simulink model "Q2_model"  (R2019a)
settings: Solver=VariableStepAuto  StartTime=0.0  StopTime=3  RelTol=1e-3
libraries: dspsigops x3
settings Model: Creator=Admin  LastModifiedBy=Admin

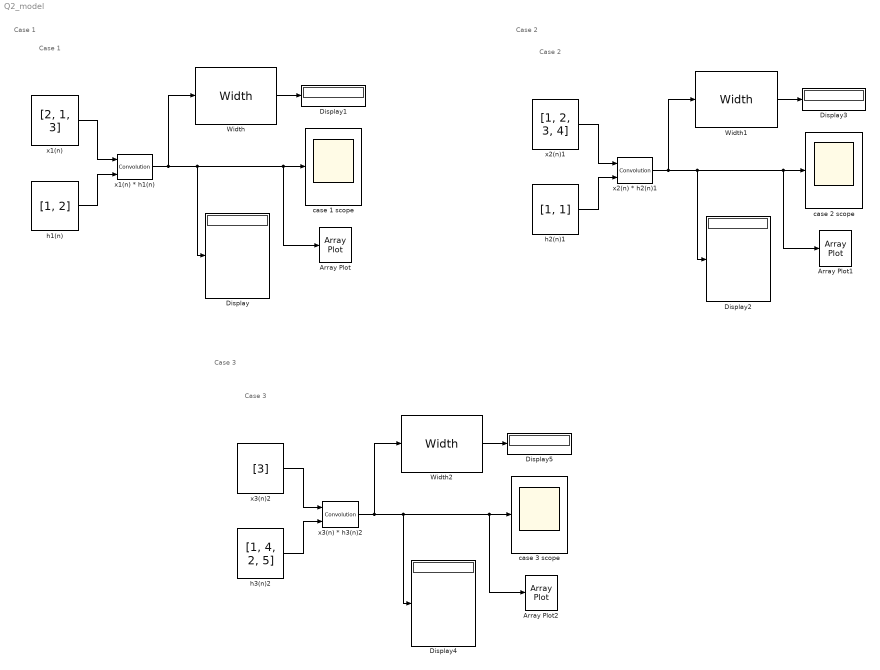
== system Q2_model ==
  note: Case 1
  note: Case 1
  note: Case 2
  note: Case 2
  note: Case 3
  note: Case 3
  Array Plot : ArrayPlot
  Array Plot1 : ArrayPlot
  Array Plot2 : ArrayPlot
  Display{,1..5} (6 alike) : Display
  Width : Width
  Width1 : Width
  Width2 : Width
  case 1 scope : Scope
  case 2 scope : Scope
  case 3 scope : Scope
  h1(n) : Constant  Value=[1, 2]  SampleTime=1
  h2(n)1 : Constant  Value=[1, 1]  SampleTime=1
  h3(n)2 : Constant  Value=[1, 4, 2, 5]  SampleTime=1
  x1(n) : Constant  Value=[2, 1, 3]  SampleTime=1
  x1(n) * h1(n) : dspsigops/Convolution  domain=Time  roundingMode=Floor  overflowMode=off  outputDataTypeStr=Inherit: Same as accumulator  outputMin=[]  outputMax=[]  outputLastDataTypeStr=Inherit: Same as accumulator
      settings: SourceProductName=DSP System Toolbox  SourceProductBaseCode=DS
  x2(n) * h2(n)1 : dspsigops/Convolution  domain=Time  roundingMode=Floor  overflowMode=off  outputDataTypeStr=Inherit: Same as accumulator  outputMin=[]  outputMax=[]  outputLastDataTypeStr=Inherit: Same as accumulator
      settings: SourceProductName=DSP System Toolbox  SourceProductBaseCode=DS
  x2(n)1 : Constant  Value=[1, 2, 3, 4]  SampleTime=1
  x3(n) * h3(n)2 : dspsigops/Convolution  domain=Time  roundingMode=Floor  overflowMode=off  outputDataTypeStr=Inherit: Same as accumulator  outputMin=[]  outputMax=[]  outputLastDataTypeStr=Inherit: Same as accumulator
      settings: SourceProductName=DSP System Toolbox  SourceProductBaseCode=DS
  x3(n)2 : Constant  Value=[3]  SampleTime=1
  wires:
  x1(n)/1 -> x1(n) * h1(n)/1
  h1(n)/1 -> x1(n) * h1(n)/2
  x1(n) * h1(n)/1 -> Display/1, case 1 scope/1, Array Plot/1, Width/1
  Width/1 -> Display1/1
  Width1/1 -> Display3/1
  x2(n) * h2(n)1/1 -> Width1/1, Array Plot1/1, case 2 scope/1, Display2/1
  h2(n)1/1 -> x2(n) * h2(n)1/2
  x2(n)1/1 -> x2(n) * h2(n)1/1
  x3(n) * h3(n)2/1 -> Width2/1, Array Plot2/1, case 3 scope/1, Display4/1
  x3(n)2/1 -> x3(n) * h3(n)2/1
  Width2/1 -> Display5/1
  h3(n)2/1 -> x3(n) * h3(n)2/2
